simulink model "t_drone"  (R2025b)
settings: Solver=ode23t  StartTime=0.0  StopTime=timespot_spl(end)+2  FixedStep=0.01  MaxStep=1e-2  MinStep=1e-13  RelTol=1e-3  AbsTol=1e-3
InitFcn:
  | model = gcs;
  | 
  | configs = evalin('base', get_param([model '/Configurations'], 'Value'));
  | hold_time = evalin('base', get_param([model '/Hold Time'], 'Value'));
  | transistion_time = evalin('base', get_param([model '/Transistion Time'], 'Value'));
  | 
  | if exist('transforms', 'var') == 1
  |     transforms = transforms;
  | else
  |     transforms = false;
  | end
  | 
  | set_drone_configurations
model workspace (MATLAB code in the model file):
  | load('xy_data_membrane.mat');
undefined symbols (not defined in the file): air_rho, battery, drone_leg, filtD_altitude, filtD_attitude, filtD_motor, filtD_pitch, filtD_position, filtD_roll, filtD_yaw, filtM_altitude, filtM_attitude, filtM_pitch, filtM_position, filtM_roll, filtM_yaw, filtSpd_motor, kd_altitude, kd_attitude, kd_motor, kd_pitch, kd_position, kd_roll, kd_yaw, ki_altitude, ki_attitude, ki_motor, ki_pitch, ki_position, ki_roll, ki_yaw, kp_altitude, kp_attitude, kp_motor, kp_pitch, kp_position, kp_roll, kp_yaw, limit_altitude, limit_attitude, limit_motor, limit_pitch, limit_roll, limit_yaw, mass, pkgDensity, pkgSize, planedepth, pos2attitude, propeller, qc_motor, qd_area, qd_drag, spline_data, spline_yaw, timespot_spl, timespots, waypoints, wind_speed, X ... (+2)
libraries: sm_lib x176, nesl_utility x46, fl_lib x37, slpidlib x9, ee_lib x5, simulink_extras x4, sdl_lib x4, simulink x2, batteryecm_lib x1
(part 1 of 8)
CloseFcn:
  | try,close(h1_quadcopter_package_delivery),end
  | clear h1_quadcopter_package_delivery
  | try,close(h2_quadcopter_package_delivery),end
  | clear h2_quadcopter_package_delivery
  | try,close(h3_quadcopter_package_delivery),end
  | clear h3_quadcopter_package_delivery
  | try,close(h4_quadcopter_package_delivery),end
  | clear h4_quadcopter_package_delivery
Description:
  | Quadcopter Package Delivery
  | Copyright 2021-2025 The MathWorks, Inc.
settings Model: VariantFading=off  Creator=tianwang  LastModifiedBy=Admin
settings SolverCC: AutoScaleAbsTol=off  MaxConsecutiveMinStep=100  AlgebraicLoopSolver=TrustRegion  SolverResetMethod=Robust
settings DataIOCC: MaxDataPoints=10000  ReturnWorkspaceOutputs=off  SignalLoggingName=logsout_quadcopter_package_delivery
settings OptimizationCC: ReuseModelBlockBuffer=off
settings DebuggingCC: ParameterPrecisionLossMsg=none  UnconnectedInputMsg=warning  UnconnectedOutputMsg=warning  UnconnectedLineMsg=warning
settings ModelReferenceCC: EnableRefExpFcnMdlSchedulingChecks=on
settings SFSimCC: CustomCodeUndefinedFunction=UseInterfaceOnly
settings RTWCC: GPUComputeCapability=3.5  DLArmComputeVersion=19.05
settings SimscapeCC: ExplicitSolverDiagnosticOptions=none  SimscapeLogType=all  SimscapeLogSimulationStatistics=on  SimscapeLogToSDI=on  SimscapeLogName=simlog_quadcopter_package_delivery  SimscapeLogLimitData=off  SimscapeLogDataHistory=50000.0
settings DiagnosticsConfigSet: SimMechanicsConflictingReferenceFrames=none  SimMechanicsRigidlyBoundBlock=none
settings ExplorerConfigSet: InternalSimMechanicsExplorerSettings=|
  | <ExplorerConfiguration>
  | 
  |   <canonicalview>default</canonicalview>
  | 
  |   <TilePanel>
  |     <TileInfo>
  |       <Tiles Columns="2" Count="4" Height="692" Rows="2" Width="984">
  |         <Row Weight="0.3531"/>
  |         <Row Weight="0.6469"/>
  |         <Column Weight="0.5664"/>
  |         <Column Weight="0.4336"/>
  |         <Tile Height="1" Width="1" X="0" Y="0"/>
  |         <Tile Height="1" Width="1" X="0" Y="1"/>
  |         <Tile Height="1" Width="1" X="1" Y="0"/>
  |         <Tile Height="1" Width="1" X="1" Y="1"/>
  |       </Tiles>
  |     </TileInfo>
  |     <SceneInfo>
  |       <SceneViewer>
  |         <IsThisViewStd>
  |           <IsStandardView>off</IsStandardView>
  |           <StandardViewName>Front</StandardViewName>
  |         </IsThisViewStd>
  |         <BGColor>
  |           <R>1</R>
  |           <G>1</G>
  |           <B>1</B>
  |           <A>1</A>
  |         </BGColor>
  |         <Camera>
  |           <DoPerspective>on</DoPerspective>
  |           <Position>
  |             <X>3.0099100000000001</X>
  |             <Y>2.9750999999999999</Y>
  |             <Z>0.14957999999999999</Z>
  |           </Position>
  |           <Center>
  |             <X>3.0099100000000001</X>
  |             <Y>3.9750999999999999</Y>
  |             <Z>0.14957999999999999</Z>
  |           </Center>
  |           <Up>
  |             <X>0</X>
  |             <Y>0</Y>
  |             <Z>1</Z>
  |           </Up>
  |           <XLim>0.46630765815499858</XLim>
  |           <YLim>0.46630765815499858</YLim>
  |           <ViewLimDist>0.01</ViewLimDist>
  |         </Camera>
  |       </SceneViewer>
  |       <SceneViewer>
  |         <IsThisViewStd>
  |           <IsStandardView>off</IsStandardView>
  |           <StandardViewName>Front</StandardViewName>
  |         </IsThisViewStd>
  |         <BGColor>
  |           <R>1</R>
  |           <G>1</G>
  |           <B>1</B>
  |           <A>1</A>
  |         </BGColor>
  |         <Camera>
  |           <DoPerspective>on</DoPerspective>
  |           <Position>
  |             <X>3.0099100000000001</X>
  |             <Y>3.9750999999999999</Y>
  |             <Z>1.14958</Z>
  |           </Position>
  |           <Center>
  |             <X>3.0099100000000001</X>
  |             <Y>3.9750999999999999</Y>
  |             <Z>0.14957999999999999</Z>
  |           </Center>
  |           <Up>
  |             <X>0</X>
  |             <Y>1</Y>
  |             <Z>0</Z>
  |           </Up>
  |           <XLim>0.46630765815499869</XLim>
  |           <YLim>0.46630765815499869</YLim>
  |           <ViewLimDist>0.01</ViewLimDist>
  |         </Camera>
  |       </SceneViewer>
  |       <SceneViewer>
  |         <IsThisViewStd>
  |           <IsStandardView>off</IsStandardView>
  |           <StandardViewName>Front</StandardViewName>
  |         </IsThisViewStd>
  |         <BGColor>
  |           <R>1</R>
  |           <G>1</G>
  |           <B>1</B>
  |           <A>1</A>
  |         </BGColor>
  |         <Camera>
  |           <DoPerspective>on</DoPerspective>
  |           <Position>
  |             <X>3.0133399999999999</X>
  |             <Y>4.0542999999999996</Y>
  |             <Z>0.21107000000000001</Z>
  |           </Position>
  |           <Center>
  |             <X>3.04318</X>
  |             <Y>5.0538499999999997</Y>
  |             <Z>0.21099999999999999</Z>
  |           </Center>
  |           <Up>
  |             <X>9.6937670845227242e-06</X>
  |             <Y>6.9742121771481852e-05</Y>
  |             <Z>0.99999999752103363</Z>
  |           </Up>
  |           <XLim>0.46630765815499881</XLim>
  |           <YLim>0.46630765815499881</YLim>
  |           <ViewLimDist>0.01</ViewLimDist>
  |         </Camera>
  |       </SceneViewer>
  |       <SceneViewer>
  |         <IsThisViewStd>
  |           <IsStandardView>off</IsStandardView>
  |           <StandardViewName>Front</StandardViewName>
  |         </IsThisViewStd>
  |         <BGColor>
  |           <R>1</R>
  |           <G>1</G>
  |           <B>1</B>
  |           <A>1</A>
  |         </BGColor>
  |         <Camera>
  |           <DoPerspective>on</DoPerspective>
  |           <Position>
  |             <X>3.5099100000000001</X>
  |             <Y>2.9750999999999999</Y>
  |             <Z>1.14958</Z>
  |           </Position>
  |           <Center>
  |             <X>3.17658</X>
  |             <Y>3.6417600000000001</Y>
  |             <Z>0.48291000000000001</Z>
  |           </Center>
  |           <Up>
  |             <X>-0.29814488151994684</X>
  |             <Y>0.59628976303989367</Y>
  |             <Z>0.74535102342271209</Z>
  |           </Up>
  |           <XLim>0.46630765815499842</XLim>
  |           <YLim>0.46630765815499842</YLim>
  |           <ViewLimDist>0.01</ViewLimDist>
  |         </Camera>
  |       </SceneViewer>
  |     </SceneInfo>
  |   </TilePanel>
  | 
  |   <MechEditorPanel>
  |     <GfxPanelCameraMap>
  |       <MapElement CameraMLId="Camera2" GfxPanelIndex="0"/>
  |       <MapElement CameraMLId="Camera1" GfxPanelIndex="1"/>
  |       <MapElement CameraMLId="Camera6" GfxPanelIndex="2"/>
  |       <MapElement CameraMLId="Camera4" GfxPanelIndex="3"/>
  |     </GfxPanelCameraMap>
  |     <Cameras>
  |       <Camera>
  |         <Id>Camera1</Id>
  |         <Value>
  |           <Name>FixO Top</Name>
  |           <NativeCamera>
  |             <PositionTrackingFeature>Quadcopter.Camera.Cam_FixO_Top.R</PositionTrackingFeature>
  |             <CenterTrackingFeature>Quadcopter.Camera.Cam_FixO_Top.R</CenterTrackingFeature>
  |             <UpVectorTrackingFeature>Quadcopter.Camera.Cam_FixO_Top.R</UpVectorTrackingFeature>
  |             <CenterTrackingOrigin>off</CenterTrackingOrigin>
  |             <CenterTrackingDirection>+X</CenterTrackingDirection>
  |             <UpVectorTrackingDirection>+Y</UpVectorTrackingDirection>
  |           </NativeCamera>
  |         </Value>
  |       </Camera>
  |       <Camera>
  |         <Id>Camera2</Id>
  |         <Value>
  |           <Name>FixO L</Name>
  |           <NativeCamera>
  |             <PositionTrackingFeature>Quadcopter.Camera.Cam_FixO_L.R</PositionTrackingFeature>
  |             <CenterTrackingFeature>Quadcopter.Camera.Cam_FixO_L.R</CenterTrackingFeature>
  |             <UpVectorTrackingFeature>Quadcopter.Camera.Cam_FixO_L.R</UpVectorTrackingFeature>
  |             <CenterTrackingOrigin>off</CenterTrackingOrigin>
  |             <CenterTrackingDirection>+X</CenterTrackingDirection>
  |             <UpVectorTrackingDirection>+Z</UpVectorTrackingDirection>
  |           </NativeCamera>
  |         </Value>
  |       </Camera>
  |       <Camera>
  |         <Id>Camera3</Id>
  |         <Value>
  |           <Name>FixO F</Name>
  |           <NativeCamera>
  |             <PositionTrackingFeature>Quadcopter.Camera.Cam_FixO_F.R</PositionTrackingFeature>
  |             <CenterTrackingFeature>Quadcopter.Camera.Cam_FixO_F.R</CenterTrackingFeature>
  |             <UpVectorTrackingFeature>Quadcopter.Camera.Cam_FixO_F.R</UpVectorTrackingFeature>
  |             <CenterTrackingOrigin>off</CenterTrackingOrigin>
  |             <CenterTrackingDirection>+X</CenterTrackingDirection>
  |             <UpVectorTrackingDirection>+Z</UpVectorTrackingDirection>
  |           </NativeCamera>
  |         </Value>
  |       </Camera>
  |       <Camera>
  |         <Id>Camera4</Id>
  |         <Value>
  |           <Name>FixO UFL</Name>
  |           <NativeCamera>
  |             <PositionTrackingFeature>Quadcopter.Camera.Cam_FixO_UFL.R</PositionTrackingFeature>
  |             <CenterTrackingFeature>Quadcopter.Camera.Cam_FixO_UFL.R</CenterTrackingFeature>
  |             <UpVectorTrackingFeature>Quadcopter.Camera.Cam_FixO_UFL.R</UpVectorTrackingFeature>
  |             <CenterTrackingOrigin>off</CenterTrackingOrigin>
  |             <CenterTrackingDirection>+X</CenterTrackingDirection>
  |             <UpVectorTrackingDirection>+Z</UpVectorTrackingDirection>
  |           </NativeCamera>
  |         </Value>
  |       </Camera>
  |       <Camera>
  |         <Id>Camera5</Id>
  |         <Value>
  |           <Name>Track_Target</Name>
  |           <NativeCamera>
  |             <PositionTrackingFeature>Quadcopter.Camera.Cam_Target.R</PositionTrackingFeature>
  |             <CenterTrackingFeature>Quadcopter.Camera.Transform_Target.F</CenterTrackingFeature>
  |             <UpVectorTrackingFeature>Quadcopter.Camera.Transform_Target.F</UpVectorTrackingFeature>
  |             <CenterTrackingOrigin>on</CenterTrackingOrigin>
  |             <UpVectorTrackingDirection>+Z</UpVectorTrackingDirection>
  |           </NativeCamera>
  |         </Value>
  |       </Camera>
  |       <Camera>
  |         <Id>Camera6</Id>
  |         <Value>
  |           <Name>Track Body Forward</Name>
  |           <NativeCamera>
  |             <PositionTrackingFeature>Quadcopter.Body.Body.Cam_Body_Front.R</PositionTrackingFeature>
  |             <CenterTrackingFeature>Quadcopter.Body.Body.Cam_Body_Front.R</CenterTrackingFeature>
  |             <UpVectorTrackingFeature>Quadcopter.Body.Body.Cam_Body_Front.R</UpVectorTrackingFeature>
  |             <CenterTrackingOrigin>off</CenterTrackingOrigin>
  |             <CenterTrackingDirection>+X</CenterTrackingDirection>
  |             <UpVectorTrackingDirection>+Z</UpVectorTrackingDirection>
  |           </NativeCamera>
  |         </Value>
  |       </Camera>
  |     </Cameras>
  |     <VideoCreator>
  |       <IncludeTiles>All</IncludeTiles>
  |       <IncludeTime>on</IncludeTime>
  |       <IncludeWorldFrame>off</IncludeWorldFrame>
  |       <PlaybackSpeedRatio>1</PlaybackSpeedRatio>
  |       <FrameRate>60</FrameRate>
  |       <FrameSize>[1920, 1080]</FrameSize>
  |       <VideoFormat>UncompressedAVI</VideoFormat>
  |     </VideoCreator>
  |   </MechEditorPanel>
  | 
  |   <PlaybackSettings>
  |     <PlaybackSpeedFactor>2</PlaybackSpeedFactor>
  |   </PlaybackSettings>
  | 
  | </ExplorerConfiguration>

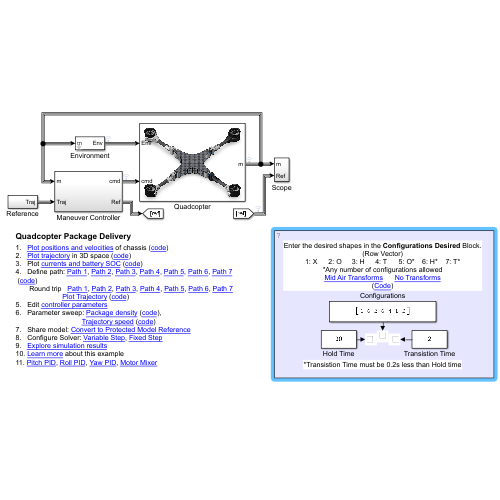
[thumbnail: Simulink's stored preview of the top-level diagram]
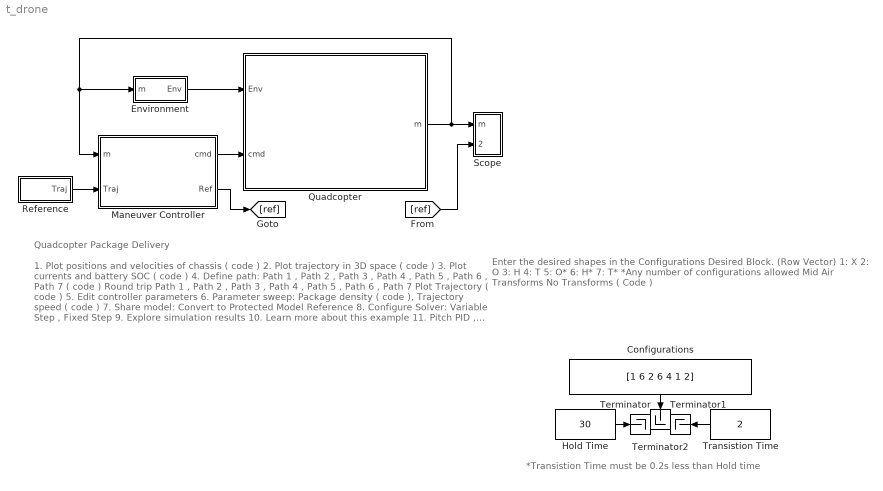
== system t_drone ==
  note: *Transistion Time must be 0.2s less than Hold time
  note: Enter the desired shapes in the Configurations Desired Block.
      | (Row Vector)
      | 1: X 2: O 3: H 4: T 5: O* 6: H* 7: T*
      | *Any number of configurations allowed
      | Mid Air Transforms No Transforms
      | ( Code )
  note: Quadcopter Package Delivery
  note: 1. Plot positions and velocities of chassis ( code )
      | 2. Plot trajectory in 3D space ( code )
      | 3. Plot currents and battery SOC ( code )
      | 4. Define path: Path 1 , Path 2 , Path 3 , Path 4 , Path 5 , Path 6 , Path 7
      | ( code )
      | Round trip Path 1 , Path 2 , Path 3 , Path 4 , Path 5 , Path 6 , Path 7
      | Plot Trajectory ( code )
      | 5. Edit controller parameters
      | 6. Parameter sweep: Package density ( code ),
      | Trajectory speed ( code )
      | 7. Share model: Convert to Protected Model Reference
      | 8. Configure Solver: Variable Step , Fixed Step
      | 9. Explore simulation results
      | 10. Learn more about this example
      | 11. Pitch PID , Roll PID , Yaw PID , Motor Mixer
  Configurations : Constant  Value=[1 6 2 6 4 1 2]
  Environment : Subsystem  mask{wind_speed_mag=wind_speed, height_max_wind=6, height_min_wind=2}
      mask prompts: wind_speed_mag "Wind Speed for Gust (m/s)"; height_max_wind "Lowest Height for Max Wind (m)"; height_min_wind "Maximum Height for Zero Wind (m)"
  Hold Time : Constant  Value=30
  Maneuver Controller : Subsystem
  Quadcopter : Subsystem
      mask Display:
      | %image('quadcopter_body_arms_load.png');
      | image('quadcopter_body_arms_load_basket.png');
  Reference : Subsystem
  Scope : Subsystem
  Terminator : Terminator
  Terminator1 : Terminator
  Terminator2 : Terminator
  Transistion Time : Constant  Value=2
  wires:
  Maneuver Controller/1(cmd) -> Quadcopter/2(cmd)
  Quadcopter/1(m) -> Maneuver Controller/1(m), Environment/1(m), Scope/1(m)
  Reference/1(Traj) -> Maneuver Controller/2(Traj)
  [ref] -> Scope/2(Ref)
  Maneuver Controller/2(Ref) -> [ref]
  Environment/1(Env) -> Quadcopter/1(Env)
  Hold Time/1 -> Terminator/1
  Transistion Time/1 -> Terminator1/1
  Configurations/1 -> Terminator2/1

== system t_drone/Environment ==
  In Bus Element : Inport  PortName=m  Element=Chassis.pz
  Bias Height Min Wind : Bias  Bias=-height_min_wind  SaturateOnIntegerOverflow=off
  Bus Creator2 : BusCreator  Inputs=1
  Constant1 : Constant  Value=0
  Mux1 : Mux  Inputs=3
  Product1 : Product
  Pulse Generator2 : DiscretePulseGenerator  PulseType=Time based  Amplitude=wind_speed_mag  Period=10  PulseWidth=25  PhaseDelay=5
  Pulse Generator3 : DiscretePulseGenerator  PulseType=Time based  Amplitude=wind_speed_mag  Period=10  PulseWidth=25  PhaseDelay=9
  Saturation : Saturate  UpperLimit=height_max_wind-height_min_wind  LowerLimit=0  ZeroCross=off
  "Scale Wind by Height " : Gain  Gain=1/(height_max_wind-height_min_wind)
  Vec to Bus : Subsystem
  Env : Outport
  wires:
  In Bus Element/1 -> Bias Height Min Wind/1
  Bias Height Min Wind/1 -> Saturation/1
  Saturation/1 -> "Scale Wind by Height "/1
  "Scale Wind by Height "/1 -> Product1/1
  Constant1/1 -> Mux1/3  "vz"
  Pulse Generator3/1 -> Mux1/2  "vy"
  Pulse Generator2/1 -> Mux1/1  "vx"
  Mux1/1 -> Product1/2  "wind"
  Product1/1 -> Vec to Bus/1(V)  "wind"
  Vec to Bus/1(B) -> Bus Creator2/1
  Bus Creator2/1 -> Env/1  "Env"

== system t_drone/Maneuver Controller ==
  In Bus Element13 : Inport  PortName=m
  In Bus Element3 : Inport  Port=2  PortName=Traj
  Altitude and YPR Control : Subsystem  mask{attitude_filtM=filtM_attitude, attitude_kp=kp_attitude, attitude_ki=ki_attitude, attitude_kd=kd_attitude, attitude_f=filtD_attitude, attitude_limit=limit_attitude, yaw_filtM=filtM_yaw, yaw_kp=kp_yaw, yaw_ki=ki_yaw, yaw_kd=kd_yaw, yaw_f=filtD_yaw, yaw_limit=limit_yaw, altitude_filtM=filtM_altitude, altitude_kp=kp_altitude, altitude_ki=ki_altitude, altitude_kd=kd_altitude, altitude_f=filtD_altitude, altitude_limit=limit_altitude}
      mask prompts: attitude_filtM "Filter Measurement (s)"; attitude_kp "Kp"; attitude_ki "Ki"; attitude_kd "Kd"; attitude_f "Derivative Filter Coefficient"; attitude_limit "Limit (m/s)"; yaw_filtM "Filter Measurement (s)"; yaw_kp "Kp"; yaw_ki "Ki"; yaw_kd "Kd"; yaw_f "Derivative Filter Coefficient"; yaw_limit "Limit (m/s)"; altitude_filtM "Filter Measurement (s)"; altitude_kp "Kp"; altitude_ki "Ki"; altitude_kd "Kd"; altitude_f "Derivative Filter Coefficient"; altitude_limit "Limit (m/s)"
      mask DialogControl Container3 Prompt: Attitude (Orientation)
      mask DialogControl Container4 Prompt: Yaw
      mask DialogControl Container_alt Prompt: Altitude (Orientation)
  Motor Mixer : Subsystem
  Position Control : Subsystem  mask{filt_pos4attitude=filtM_position, kp_xy2ypr=kp_position, ki_xy2ypr=ki_position, kd_xy2ypr=kd_position, filtD_xy2ypr=filtD_position, err2rp=pos2attitude}
      mask prompts: filt_pos4attitude "Filter Constant (s)"; kp_xy2ypr "Kp"; ki_xy2ypr "Ki"; kd_xy2ypr "Kd"; filtD_xy2ypr "Derivative Filter Coefficient"; err2rp "Position Error to Attitude"
  cmd : Outport
  Ref : Outport  Port=2
  wires:
  Motor Mixer/1(Cmd) -> cmd/1
  Altitude and YPR Control/2(Motor Roll) -> Motor Mixer/2(Roll Cmd)
  Altitude and YPR Control/1(Motor Pitch) -> Motor Mixer/1(Pitch Cmd)
  Altitude and YPR Control/3(Motor Yaw) -> Motor Mixer/3(Yaw Cmd)
  Altitude and YPR Control/4(Motor Thrust) -> Motor Mixer/4(Thrust Cmd)
  Position Control/2(Roll Cmd) -> Altitude and YPR Control/4(Roll Cmd)
  Position Control/1(Pitch Cmd) -> Altitude and YPR Control/3(Pitch Cmd)
  In Bus Element13/1 -> Position Control/1(m), Altitude and YPR Control/1(m)
  In Bus Element3/1 -> Position Control/2(Traj), Altitude and YPR Control/2(Ref)
  Position Control/3(Yaw Cmd) -> Altitude and YPR Control/5(Yaw Cmd)
  Position Control/4(Ref) -> Ref/1

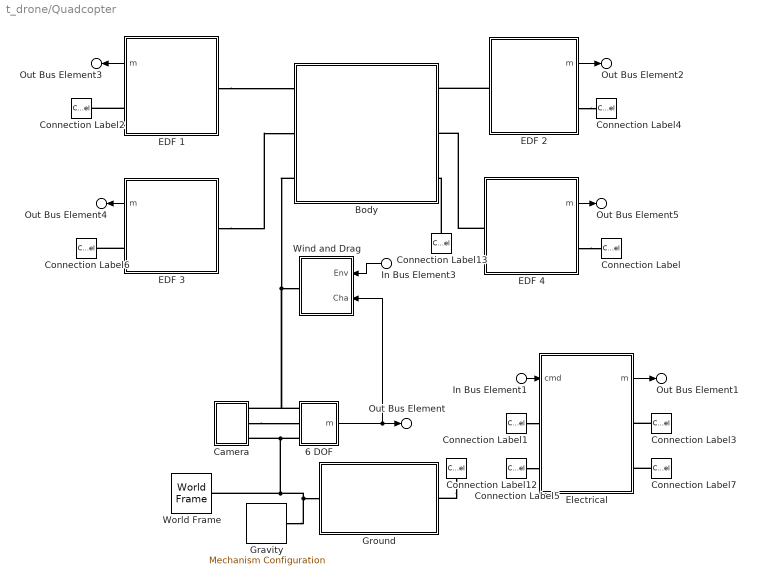
== system t_drone/Quadcopter ==
  In Bus Element3 : Inport  PortName=Env  Element=wind
  In Bus Element1 : Inport  Port=2  PortName=cmd
  6 DOF : Subsystem
  Body : Subsystem
      mask Display: image('quadcopter_body_arms.png');
  Camera : Subsystem
  Connection Label : ConnectionLabel  Label=P4
  Connection Label1 : ConnectionLabel  Label=P4
  Connection Label12 : ConnectionLabel  Label=G
  Connection Label13 : ConnectionLabel  Label=G
  Connection Label2 : ConnectionLabel  Label=P1
  Connection Label3 : ConnectionLabel  Label=P1
  Connection Label4 : ConnectionLabel  Label=P2
  Connection Label5 : ConnectionLabel  Label=P2
  Connection Label6 : ConnectionLabel  Label=P3
  Connection Label7 : ConnectionLabel  Label=P3
  EDF 1 : Subsystem  mask{popup_prop_pos=1 or 4}
      mask prompts: popup_prop_pos "Propeller Position"
      mask init:
      | if(strcmp(get_param(gcb,'popup_prop_pos'),'1 or 4'))
      |     set_param([gcb '/Propeller'],'ExtGeomFileName','quadcopter_drone_12_blade_fans.stp');
      |     set_param([gcb '/Thrust Direction'],'Gain','1');
      | else
      |     set_param([gcb '/Propeller'],'ExtGeomFileName','quadcopter_drone_12_blade_fans.stp');
      |     set_param([gcb '/Thrust Direction'],'Gain','-1');
      | end
      mask TypeOptions popup_prop_pos: 1 or 4 | 2 or 3
      mask Display:
      | if(strcmp(get_param(gcb,'popup_prop_pos'),'1 or 4'))
      |     image('quadcopter_motor_prop_1_4.png');
      | else
      |     image('quadcopter_motor_prop_2_3.png');
      | end
  EDF 2 : Subsystem  mask{popup_prop_pos=2 or 3}
      mask prompts: popup_prop_pos "Propeller Position"
      mask init: same as t_drone/Quadcopter/EDF 1
      mask TypeOptions popup_prop_pos: 1 or 4 | 2 or 3
      mask Display:
      | if(strcmp(get_param(gcb,'popup_prop_pos'),'1 or 4'))
      |     image('quadcopter_motor_prop_1_4.png');
      | else
      |     image('quadcopter_motor_prop_2_3.png');
      | end
  EDF 3 : Subsystem  mask{popup_prop_pos=2 or 3}
      mask prompts: popup_prop_pos "Propeller Position"
      mask init: same as t_drone/Quadcopter/EDF 1
      mask TypeOptions popup_prop_pos: 1 or 4 | 2 or 3
      mask Display:
      | if(strcmp(get_param(gcb,'popup_prop_pos'),'1 or 4'))
      |     image('quadcopter_motor_prop_1_4.png');
      | else
      |     image('quadcopter_motor_prop_2_3.png');
      | end
  EDF 4 : Subsystem  mask{popup_prop_pos=1 or 4}
      mask prompts: popup_prop_pos "Propeller Position"
      mask init: same as t_drone/Quadcopter/EDF 1
      mask TypeOptions popup_prop_pos: 1 or 4 | 2 or 3
      mask Display:
      | if(strcmp(get_param(gcb,'popup_prop_pos'),'1 or 4'))
      |     image('quadcopter_motor_prop_1_4.png');
      | else
      |     image('quadcopter_motor_prop_2_3.png');
      | end
  Electrical : Subsystem  mask{trq_max=qc_motor.max_torque, power_max=qc_motor.max_power, trq_tc=qc_motor.time_const, eff_overall=qc_motor.efficiency, eff_spd=qc_motor.efficiency_spd, eff_trq=qc_motor.efficiency_trq, rotor_d=qc_motor.rotor_damping, kp=kp_motor, ki=ki_motor, kd=kd_motor, f_deriv=filtD_motor, f_spd=filtSpd_motor, max_trq_cmd=limit_motor}
      mask prompts: trq_max "Max Torque (N*m)"; power_max "Max Power (W)"; trq_tc "Time Constant, Torque (s)"; eff_overall "Efficiency (%)"; eff_spd "Speed for Efficiency (rpm)"; eff_trq "Torque for Efficiency (N*m)"; rotor_d "Rotor Damping (N*m/(rad/s))"; kp "Proportional"; ki "Integral"; kd "Derivative"; f_deriv "Filter on Error Derivative (N)"; f_spd "Filter on Speed Measurement (sec)"; max_trq_cmd "Saturation (N*m)"
      mask DialogControl Container4 Prompt: Motor
      mask DialogControl Container9 Prompt: Control
      mask Display: image('quadcopter_electric.png');
  Gravity : sm_lib/Utilities/Mechanism Configuration  UniformGravity=Constant  GravityVector=[0 0 -9.80665]  GravityVectorUnits=m/s^2  LinearizationDelta=0.001  JointModeTransitionNonlinearIterations=2
  Ground : Subsystem
      mask Display: image('ground_launch_target.PNG');
  Wind and Drag : Subsystem
  World Frame : sm_lib/Frames and Transforms/World Frame
  Out Bus Element : Outport  PortName=m  Element=Chassis
  Out Bus Element1 : Outport  PortName=m  Element=Motor
  Out Bus Element2 : Outport  PortName=m  Element=Prop2
  Out Bus Element3 : Outport  PortName=m  Element=Prop1
  Out Bus Element4 : Outport  PortName=m  Element=Prop3
  Out Bus Element5 : Outport  PortName=m  Element=Prop4
  wires:
  EDF 4/1(m) -> Out Bus Element5/1
  EDF 1/1(m) -> Out Bus Element3/1
  EDF 3/1(m) -> Out Bus Element4/1
  Electrical/1(m) -> Out Bus Element1/1
  EDF 2/1(m) -> Out Bus Element2/1
  In Bus Element1/1 -> Electrical/1(cmd)
  6 DOF/1(m) -> Out Bus Element/1, Wind and Drag/2(Cha)
  In Bus Element3/1 -> Wind and Drag/1(Env)
  connections:
  Body/LConn3 -- 6 DOF/LConn1 -- Camera/RConn1 -- Wind and Drag/RConn1
  EDF 2/LConn1 -- Body/RConn1
  EDF 1/LConn1 -- Body/LConn1
  EDF 4/LConn1 -- Body/RConn2
  EDF 3/LConn1 -- Body/LConn2
  Connection Label13/LConn1 -- Body/RConn3
  EDF 4/RConn1 -- Connection Label/LConn1
  Connection Label1/LConn1 -- Electrical/LConn1
  EDF 1/RConn1 -- Connection Label2/LConn1
  Connection Label3/LConn1 -- Electrical/RConn1
  EDF 2/RConn1 -- Connection Label4/LConn1
  Connection Label5/LConn1 -- Electrical/LConn2
  EDF 3/RConn1 -- Connection Label6/LConn1
  Connection Label7/LConn1 -- Electrical/RConn2
  Gravity/RConn1 -- 6 DOF/LConn3 -- Camera/RConn3 -- World Frame/RConn1 -- Ground/RConn1
  Connection Label12/LConn1 -- Ground/LConn1
  Camera/RConn2 -- 6 DOF/LConn2

== system t_drone/Reference ==
  Clock1 : Clock
  Derivative : Subsystem
  Interpolate Spline Points : Subsystem
  Out Bus Element : Outport  PortName=Traj  Element=pos
  Out Bus Element1 : Outport  PortName=Traj  Element=vel
  Out Bus Element2 : Outport  PortName=Traj  Element=yaw
  wires:
  Clock1/1 -> Interpolate Spline Points/1(In1)
  Interpolate Spline Points/2(des_pos) -> Out Bus Element/1, Derivative/1(des xyz)
  Interpolate Spline Points/1(Yaw) -> Out Bus Element2/1
  Derivative/1(des_vel) -> Out Bus Element1/1

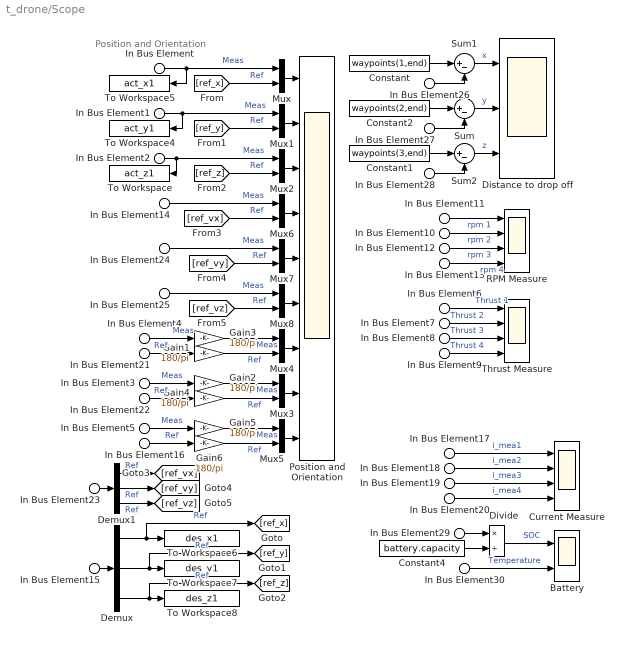
== system t_drone/Scope ==
  note: Position and Orientation
  In Bus Element : Inport  PortName=m  Element=Chassis.px
  In Bus Element26 : Inport  PortName=m  Element=Chassis.px
  In Bus Element1 : Inport  PortName=m  Element=Chassis.py
  In Bus Element27 : Inport  PortName=m  Element=Chassis.py
  In Bus Element2 : Inport  PortName=m  Element=Chassis.pz
  In Bus Element28 : Inport  PortName=m  Element=Chassis.pz
  In Bus Element3 : Inport  PortName=m  Element=Chassis.pitch
  In Bus Element4 : Inport  PortName=m  Element=Chassis.roll
  In Bus Element5 : Inport  PortName=m  Element=Chassis.yaw
  In Bus Element14 : Inport  PortName=m  Element=Chassis.vx
  In Bus Element24 : Inport  PortName=m  Element=Chassis.vy
  In Bus Element25 : Inport  PortName=m  Element=Chassis.vz
  In Bus Element7 : Inport  PortName=m  Element=Prop2.thrust
  In Bus Element10 : Inport  PortName=m  Element=Prop2.w
  In Bus Element6 : Inport  PortName=m  Element=Prop1.thrust
  In Bus Element11 : Inport  PortName=m  Element=Prop1.w
  In Bus Element8 : Inport  PortName=m  Element=Prop3.thrust
  In Bus Element12 : Inport  PortName=m  Element=Prop3.w
  In Bus Element9 : Inport  PortName=m  Element=Prop4.thrust
  In Bus Element13 : Inport  PortName=m  Element=Prop4.w
  In Bus Element17 : Inport  PortName=m  Element=Motor.Mot1.i
  In Bus Element18 : Inport  PortName=m  Element=Motor.Mot2.i
  In Bus Element19 : Inport  PortName=m  Element=Motor.Mot3.i
  In Bus Element20 : Inport  PortName=m  Element=Motor.Mot4.i
  In Bus Element29 : Inport  PortName=m  Element=Motor.Battery.SOC
  In Bus Element30 : Inport  PortName=m  Element=Motor.Battery.degC
  In Bus Element15 : Inport  Port=2  PortName=Ref  Element=pos
  In Bus Element16 : Inport  Port=2  PortName=Ref  Element=yaw
  In Bus Element21 : Inport  Port=2  PortName=Ref  Element=roll
  In Bus Element22 : Inport  Port=2  PortName=Ref  Element=pitch
  In Bus Element23 : Inport  Port=2  PortName=Ref  Element=vel
  Battery : Scope  NumInputPorts=2
      settings: ActiveDisplayYMinimum=0.99219  ActiveDisplayYMaximum=1.00087
  Constant : Constant  Value=waypoints(1,end)
  Constant1 : Constant  Value=waypoints(3,end)
  Constant2 : Constant  Value=waypoints(2,end)
  Constant4 : Constant  Value=battery.capacity
  Current Measure : Scope  NumInputPorts=4
      settings: ActiveDisplayYMinimum=-5.48055  ActiveDisplayYMaximum=19.1285  DataLoggingVariableName=ScopeData2
  Demux : Demux  Outputs=3
  Demux1 : Demux  Outputs=3
  Distance to drop off : Scope  NumInputPorts=3
      settings: ActiveDisplayYMinimum=-0.83846  ActiveDisplayYMaximum=0.45879
  Divide : Product  Inputs=*/
  Gain{1..6} (6 alike) : Gain  Gain=180/pi
  Mux{,1..8} (9 alike) : Mux  Inputs=2
  Position and Orientation : Scope  NumInputPorts=9
      settings: Title=px  ActiveDisplayYMinimum=-2.95256  ActiveDisplayYMaximum=5.99591  DataLoggingVariableName=ScopeData2
  RPM Measure : Scope  NumInputPorts=4
      settings: ActiveDisplayYMinimum=-7347.52347  ActiveDisplayYMaximum=7432.06356  DataLoggingVariableName=ScopeData2
  Sum : Sum  Inputs=|+-
  Sum1 : Sum  Inputs=|+-
  Sum2 : Sum  Inputs=|+-
  Thrust Measure : Scope  NumInputPorts=4
      settings: ActiveDisplayYMinimum=-0.67587  ActiveDisplayYMaximum=6.05582
  To Workspace : ToWorkspace  VariableName=act_z1  SampleTime=-1
  To Workspace4 : ToWorkspace  VariableName=act_y1  SampleTime=-1
  To Workspace5 : ToWorkspace  VariableName=act_x1  SampleTime=-1
  To Workspace6 : ToWorkspace  VariableName=des_x1  SampleTime=-1
  To Workspace7 : ToWorkspace  VariableName=des_y1  SampleTime=-1
  To Workspace8 : ToWorkspace  VariableName=des_z1  SampleTime=-1
  wires:
  In Bus Element7/1 -> Thrust Measure/2  "Thrust 2"
  In Bus Element9/1 -> Thrust Measure/4  "Thrust 4"
  In Bus Element8/1 -> Thrust Measure/3  "Thrust 3"
  In Bus Element6/1 -> Thrust Measure/1  "Thrust 1"
  In Bus Element11/1 -> RPM Measure/1  "rpm 1"
  In Bus Element10/1 -> RPM Measure/2  "rpm 2"
  In Bus Element12/1 -> RPM Measure/3  "rpm 3"
  In Bus Element13/1 -> RPM Measure/4  "rpm 4"
  Demux/3 -> [ref_z], To Workspace8/1  "Ref"
  In Bus Element2/1 -> Mux2/1, To Workspace/1  "Meas"
  In Bus Element17/1 -> Current Measure/1  "i_mea1"
  In Bus Element18/1 -> Current Measure/2  "i_mea2"
  In Bus Element19/1 -> Current Measure/3  "i_mea3"
  In Bus Element20/1 -> Current Measure/4  "i_mea4"
  Gain2/1 -> Mux3/1  "Meas"
  Gain3/1 -> Mux4/1  "Meas"
  Gain5/1 -> Mux5/1  "Meas"
  Demux/2 -> [ref_y], To Workspace7/1  "Ref"
  In Bus Element1/1 -> Mux1/1, To Workspace4/1  "Meas"
  Demux/1 -> To Workspace6/1, [ref_x]  "Ref"
  In Bus Element/1 -> Mux/1, To Workspace5/1  "Meas"
  In Bus Element28/1 -> Sum2/2
  Constant1/1 -> Sum2/1
  Constant2/1 -> Sum/1
  In Bus Element27/1 -> Sum/2
  Constant/1 -> Sum1/1
  In Bus Element26/1 -> Sum1/2
  Sum/1 -> Distance to drop off/2  "y"
  Sum1/1 -> Distance to drop off/1  "x"
  Sum2/1 -> Distance to drop off/3  "z"
  Mux/1 -> Position and Orientation/1
  Mux1/1 -> Position and Orientation/2
  Mux2/1 -> Position and Orientation/3
  Mux3/1 -> Position and Orientation/8
  Mux4/1 -> Position and Orientation/7
  Mux5/1 -> Position and Orientation/9
  In Bus Element15/1 -> Demux/1
  [ref_x] -> Mux/2  "Ref"
  [ref_y] -> Mux1/2  "Ref"
  [ref_z] -> Mux2/2  "Ref"
  In Bus Element23/1 -> Demux1/1
  Demux1/1 -> [ref_vx]  "Ref"
  Demux1/2 -> [ref_vy]  "Ref"
  Demux1/3 -> [ref_vz]  "Ref"
  Mux8/1 -> Position and Orientation/6
  Mux7/1 -> Position and Orientation/5
  Mux6/1 -> Position and Orientation/4
  [ref_vx] -> Mux6/2  "Ref"
  [ref_vy] -> Mux7/2  "Ref"
  [ref_vz] -> Mux8/2  "Ref"
  In Bus Element14/1 -> Mux6/1  "Meas"
  In Bus Element24/1 -> Mux7/1  "Meas"
  In Bus Element25/1 -> Mux8/1  "Meas"
  In Bus Element21/1 -> Gain1/1  "Ref"
  In Bus Element22/1 -> Gain4/1  "Ref"
  In Bus Element16/1 -> Gain6/1  "Ref"
  In Bus Element4/1 -> Gain3/1  "Meas"
  Gain1/1 -> Mux4/2  "Ref"
  In Bus Element3/1 -> Gain2/1  "Meas"
  Gain4/1 -> Mux3/2  "Ref"
  In Bus Element5/1 -> Gain5/1  "Meas"
  Gain6/1 -> Mux5/2  "Ref"
  In Bus Element29/1 -> Divide/1
  Constant4/1 -> Divide/2
  Divide/1 -> Battery/1  "SOC"
  In Bus Element30/1 -> Battery/2  "Temperature"

== system t_drone/Environment/Vec to Bus ==
  V : Inport
  Bus Creator : BusCreator  Inputs=3
  Demux : Demux  Outputs=3
  B : Outport
  wires:
  Demux/3 -> Bus Creator/3  "vz"
  V/1 -> Demux/1
  Demux/1 -> Bus Creator/1  "vx"
  Demux/2 -> Bus Creator/2  "vy"
  Bus Creator/1 -> B/1  "wind"

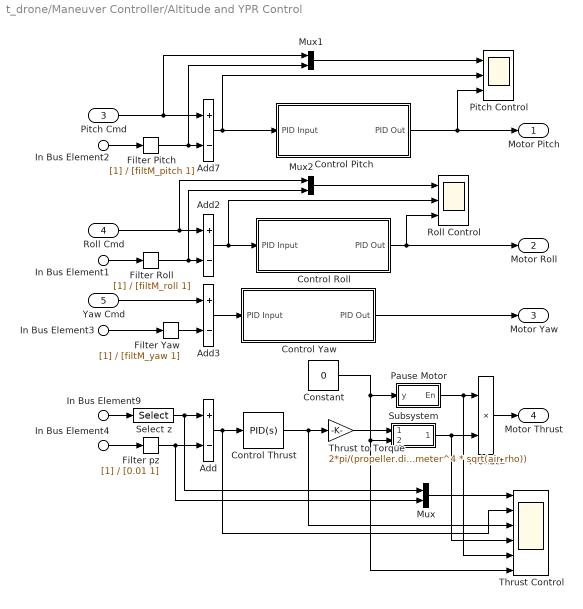
== system t_drone/Maneuver Controller/Altitude and YPR Control ==
  In Bus Element1 : Inport  PortName=m  Element=Chassis.roll
  In Bus Element2 : Inport  PortName=m  Element=Chassis.pitch
  In Bus Element3 : Inport  PortName=m  Element=Chassis.yaw
  In Bus Element4 : Inport  PortName=m  Element=Chassis.pz
  In Bus Element9 : Inport  Port=2  PortName=Ref  Element=pos
  Pitch Cmd : Inport  Port=3
  Roll Cmd : Inport  Port=4
  Yaw Cmd : Inport  Port=5
  Add{,2..3,7} (4 alike) : Sum  Inputs=+-
  Constant : Constant  Value=0
  Control Pitch : Subsystem  mask{ts_p=kp_pitch, ts_i=ki_pitch, ts_d=kd_pitch, ts_f=filtD_pitch, ts_l=limit_pitch, time_spots=timespots}
      mask prompts: ts_p "Proportional"; ts_i "Integral"; ts_d "Derivative"; ts_f "Filter Coefficient"; ts_l "Limit"; time_spots "Time Intervals"
  Control Roll : Subsystem  mask{ts_p=kp_roll, ts_i=ki_roll, ts_d=kd_roll, ts_f=filtD_roll, ts_l=limit_roll, time_spots=timespots}
      mask prompts: ts_p "Proportional"; ts_i "Integral"; ts_d "Derivative"; ts_f "Filter Coefficient"; ts_l "Limit"; time_spots "Time Intervals"
  Control Thrust : slpidlib/PID Controller  Controller=PID  Form=Parallel  TimeDomain=Continuous-time  UseExternalTs=off  SampleTime=-1  IntegratorMethod=Forward Euler  FilterMethod=Forward Euler  ControllerParametersSource=internal  P=altitude_kp  I=altitude_ki  UseKiTs=off  D=altitude_kd  UseExternalDerivativeSource=off  N=altitude_f  UseFilter=on  TunerSelectOption=Transfer Function Based (PID Tuner App)  ZeroCross=off  InitialConditionSource=internal  InitialConditionForIntegrator=0  InitialConditionForFilter=0  DifferentiatorICPrevScaledInput=0  ExternalReset=none  TrackingMode=off  Kt=1  LimitOutput=on  SatLimitsSource=internal  UpperSaturationLimit=altitude_limit  LowerSaturationLimit=-altitude_limit  LinearizeAsGain=on  AntiWindupMode=none  Kb=1  LimitIntegrator=off  UpperIntegratorSaturationLimit=inf  LowerIntegratorSaturationLimit=-inf  POutMin=[]  POutMax=[]  IOutMin=[]  IOutMax=[]  DOutMin=[]  DOutMax=[]  NOutMin=[]  NOutMax=[]  SumOutMin=[]  SumOutMax=[]  SaturationOutMin=[]  SaturationOutMax=[]  PParamMin=[]  PParamMax=[]  IParamMin=[]  IParamMax=[]  DParamMin=[]  DParamMax=[]  NParamMin=[]  NParamMax=[]  KbParamMin=[]  KbParamMax=[]  KtParamMin=[]  KtParamMax=[]  KbOutMin=[]  KbOutMax=[]  KtOutMin=[]  KtOutMax=[]  IntegratorOutMin=[]  IntegratorOutMax=[]  FilterOutMin=[]  FilterOutMax=[]  SumI1OutMin=[]  SumI1OutMax=[]  SumI2OutMin=[]  SumI2OutMax=[]  SumI3OutMin=[]  SumI3OutMax=[]  SumI4OutMin=[]  SumI4OutMax=[]  SumDOutMin=[]  SumDOutMax=[]  DifferentiatorOutMin=[]  DifferentiatorOutMax=[]  FilterDiffOutCoefMin=[]  FilterDiffOutCoefMax=[]  ReciprocalOutMin=[]  ReciprocalOutMax=[]  SumDenOutMin=[]  SumDenOutMax=[]  SumNumOutMin=[]  SumNumOutMax=[]  DivideOutMin=[]  DivideOutMax=[]  UdiffTsProdOutMin=[]  UdiffTsProdOutMax=[]  NTsProdOutMin=[]  NTsProdOutMax=[]  UintegralTsProdOutMin=[]  UintegralTsProdOutMax=[]  UngainTsProdOutMin=[]  UngainTsProdOutMax=[]  ClampingZeroOutDataTypeStr=Inherit: Inherit via back propagation  ClampingZeroOutMin=[]  ClampingZeroOutMax=[]  FilterDenConstantOutDataTypeStr=Inherit: Inherit via back propagation  FilterDenConstantOutMin=[]  FilterDenConstantOutMax=[]  PCopyOutDataTypeStr=Inherit: Inherit via back propagation  PCopyOutMin=[]  PCopyOutMax=[]  NCopyOutDataTypeStr=Inherit: Inherit via back propagation  NCopyOutMin=[]  NCopyOutMax=[]  IntegratorContinuousStateAttributes=''  IntegratorStateMustResolveToSignalObject=off  IntegratorRTWStateStorageClass=Auto  FilterContinuousStateAttributes=''  FilterStateMustResolveToSignalObject=off  FilterRTWStateStorageClass=Auto  ParallelPVariant=InternalParameters  IdealPVariant=Disabled  IVariant=InternalParameters  DVariant=InternalParameters  IntegratorVariant=Continuous  SatVariant=Enabled  AWVariant=Passthrough  PCopyVariant=Disabled  TRVariant=Disabled  FdbkBlocksVariant=Forward  IdealPFdbkVariant=Disabled  SatFdbkVariant=Disabled  DerivativeFilterVariant=ContFilter  NVariant=InternalParameters  NCopyVariant=Disabled  FilterICVariant=InternalICsFilter  IntegratorICVariant=InternalICs  ExternalResetVariant=Disabled  TRSumVariant=Passthrough  SumFdbkVariant=Disabled  SumVariant=Sum_PID  TsampFilterVariant=InternalTs  TsampNgainVariant=Passthrough  TsampIntegralVariant=Disabled_SignalSpec  ExternalSaturationOutDataTypeStr=Inherit: Same as second input  DerivativeSourceVariant=ErrorSignal  PreIntVariant=InternalPreInt
  Control Yaw : Subsystem  mask{ts_p=kp_yaw, ts_i=ki_yaw, ts_d=kd_yaw, ts_f=filtD_yaw, ts_l=limit_yaw, time_spots=timespots}
      mask prompts: ts_p "Proportional"; ts_i "Integral"; ts_d "Derivative"; ts_f "Filter Coefficient"; ts_l "Limit"; time_spots "Time Intervals"
  Filter Pitch : TransferFcn  Denominator=[filtM_pitch 1]
  Filter Roll : TransferFcn  Denominator=[filtM_roll 1]
  Filter Yaw : TransferFcn  Denominator=[filtM_yaw 1]
  Filter pz : TransferFcn  Denominator=[0.01 1]
  Mux : Mux  Inputs=2
  Mux1 : Mux  Inputs=2
  Mux2 : Mux  Inputs=2
  Pause Motor : Subsystem  mask{ts_pulse=0.5, dur_pulse=2}
      mask prompts: ts_pulse "Pulse resolution (sec)"; dur_pulse "Pulse duration (sec)"
  Pitch Control : Scope  NumInputPorts=3
      settings: ActiveDisplayYMinimum=-0.80585  ActiveDisplayYMaximum=0.83815
  Product : Product
  Roll Control : Scope  NumInputPorts=3
      settings: ActiveDisplayYMinimum=-0.80585  ActiveDisplayYMaximum=0.83815
  Select z : Selector  InputPortWidth=3  IndexOptions=Index vector (dialog)  Indices=[3]  OutputSizes=1
  Subsystem : Subsystem
  Thrust Control : Scope  NumInputPorts=6
      settings: ActiveDisplayYMinimum=-0.7525151669788791  ActiveDisplayYMaximum=6.772636502809914  DataLoggingVariableName=ScopeData2
  Thrust to Torque : Gain  Gain=2*pi/(propeller.diameter^4 * sqrt(air_rho))
  Motor Pitch : Outport
  Motor Roll : Outport  Port=2
  Motor Yaw : Outport  Port=3
  Motor Thrust : Outport  Port=4
  wires:
  Pitch Cmd/1 -> Mux1/1, Add7/1
  In Bus Element3/1 -> Filter Yaw/1
  Add7/1 -> Control Pitch/1(PID Input), Pitch Control/2
  Yaw Cmd/1 -> Add3/1
  In Bus Element2/1 -> Filter Pitch/1
  Select z/1 -> Mux/1, Add/1
  In Bus Element1/1 -> Filter Roll/1
  Add3/1 -> Control Yaw/1(PID Input)
  In Bus Element9/1 -> Select z/1
  Add/1 -> Control Thrust/1, Thrust Control/2
  Control Thrust/1 -> Thrust Control/3, Thrust to Torque/1
  Mux/1 -> Thrust Control/1
  Mux1/1 -> Pitch Control/1
  In Bus Element4/1 -> Filter pz/1
  Filter Pitch/1 -> Mux1/2, Add7/2
  Filter Yaw/1 -> Add3/2
  Filter pz/1 -> Mux/2, Add/2
  Product/1 -> Motor Thrust/1
  Pause Motor/1(En) -> Thrust Control/5, Product/1
  Constant/1 -> Pause Motor/1(y), Thrust Control/6, Subsystem/2(load)
  Subsystem/1(Out1) -> Product/2, Thrust Control/4
  Thrust to Torque/1 -> Subsystem/1(cmd)
  Filter Roll/1 -> Mux2/2, Add2/2
  Mux2/1 -> Roll Control/1
  Add2/1 -> Control Roll/1(PID Input), Roll Control/2
  Roll Cmd/1 -> Add2/1, Mux2/1
  Control Pitch/1(PID Out) -> Pitch Control/3, Motor Pitch/1
  Control Roll/1(PID Out) -> Motor Roll/1, Roll Control/3
  Control Yaw/1(PID Out) -> Motor Yaw/1

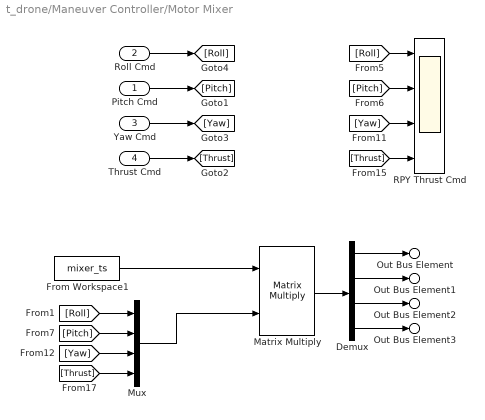
== system t_drone/Maneuver Controller/Motor Mixer ==
  Pitch Cmd : Inport
  Roll Cmd : Inport  Port=2
  Yaw Cmd : Inport  Port=3
  Thrust Cmd : Inport  Port=4
  Demux : Demux
  From Workspace1 : FromWorkspace  VariableName=mixer_ts  OutputAfterFinalValue=Holding final value
  Matrix Multiply : Product  Multiplication=Matrix(*)
  Mux : Mux
  RPY Thrust Cmd : Scope  NumInputPorts=4
      settings: ActiveDisplayYMinimum=4417.97471  ActiveDisplayYMaximum=5987.32527
  Out Bus Element : Outport  PortName=Cmd  Element=w1
  Out Bus Element1 : Outport  PortName=Cmd  Element=w2
  Out Bus Element2 : Outport  PortName=Cmd  Element=w3
  Out Bus Element3 : Outport  PortName=Cmd  Element=w4
  wires:
  Roll Cmd/1 -> [Roll]
  Pitch Cmd/1 -> [Pitch]
  Yaw Cmd/1 -> [Yaw]
  Thrust Cmd/1 -> [Thrust]
  [Roll] -> Mux/1
  [Roll] -> RPY Thrust Cmd/1
  [Pitch] -> RPY Thrust Cmd/2
  [Pitch] -> Mux/2
  [Yaw] -> RPY Thrust Cmd/3
  [Yaw] -> Mux/3
  [Thrust] -> RPY Thrust Cmd/4
  [Thrust] -> Mux/4
  Matrix Multiply/1 -> Demux/1
  Demux/1 -> Out Bus Element/1
  From Workspace1/1 -> Matrix Multiply/1
  Mux/1 -> Matrix Multiply/2
  Demux/2 -> Out Bus Element1/1
  Demux/3 -> Out Bus Element2/1
  Demux/4 -> Out Bus Element3/1

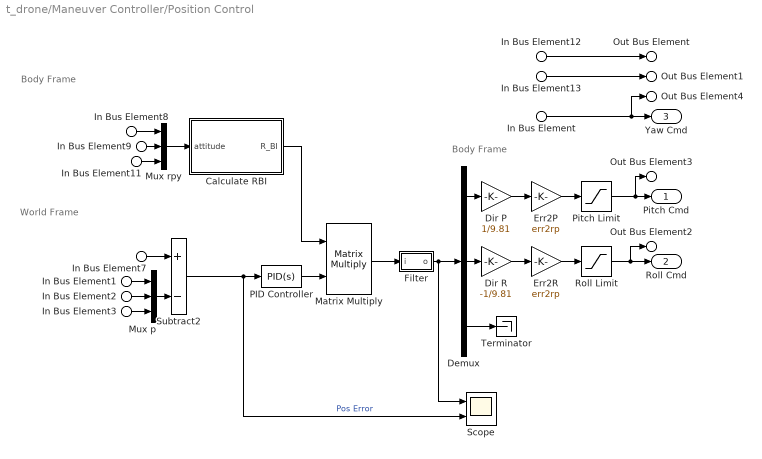
== system t_drone/Maneuver Controller/Position Control ==
  note: Body Frame
  note: World Frame
  note: Body Frame
  In Bus Element1 : Inport  PortName=m  Element=Chassis.px
  In Bus Element2 : Inport  PortName=m  Element=Chassis.py
  In Bus Element3 : Inport  PortName=m  Element=Chassis.pz
  In Bus Element8 : Inport  PortName=m  Element=Chassis.roll
  In Bus Element9 : Inport  PortName=m  Element=Chassis.pitch
  In Bus Element11 : Inport  PortName=m  Element=Chassis.yaw
  In Bus Element7 : Inport  Port=2  PortName=Traj  Element=pos
  In Bus Element12 : Inport  Port=2  PortName=Traj  Element=pos
  In Bus Element13 : Inport  Port=2  PortName=Traj  Element=vel
  In Bus Element : Inport  Port=2  PortName=Traj  Element=yaw
  Calculate RBI : MATLAB Function  TreatAsAtomicUnit=on
  Demux : Demux  Outputs=3
  Dir P : Gain  Gain=1/9.81
  Dir R : Gain  Gain=-1/9.81
  Err2P : Gain  Gain=err2rp
  Err2R : Gain  Gain=err2rp
  Filter : Subsystem  mask{filt_const=filt_pos4attitude}
      mask prompts: filt_const "Filter Constant"
  Matrix Multiply : Product  Multiplication=Matrix(*)
  Mux p : Mux  Inputs=3
  Mux rpy : Mux  Inputs=3
  PID Controller : slpidlib/PID Controller  Controller=PID  Form=Parallel  TimeDomain=Continuous-time  UseExternalTs=off  SampleTime=-1  IntegratorMethod=Forward Euler  FilterMethod=Forward Euler  ControllerParametersSource=internal  P=kp_xy2ypr  I=ki_xy2ypr  UseKiTs=off  D=kd_xy2ypr  UseExternalDerivativeSource=off  N=filtD_xy2ypr  UseFilter=on  TunerSelectOption=Transfer Function Based (PID Tuner App)  InitialConditionSource=internal  InitialConditionForIntegrator=0  InitialConditionForFilter=0  DifferentiatorICPrevScaledInput=0  ExternalReset=none  TrackingMode=off  Kt=1  LimitOutput=off  SatLimitsSource=internal  UpperSaturationLimit=inf  LowerSaturationLimit=-inf  LinearizeAsGain=on  AntiWindupMode=none  Kb=1  LimitIntegrator=off  UpperIntegratorSaturationLimit=inf  LowerIntegratorSaturationLimit=-inf  POutMin=[]  POutMax=[]  IOutMin=[]  IOutMax=[]  DOutMin=[]  DOutMax=[]  NOutMin=[]  NOutMax=[]  SumOutMin=[]  SumOutMax=[]  SaturationOutMin=[]  SaturationOutMax=[]  PParamMin=[]  PParamMax=[]  IParamMin=[]  IParamMax=[]  DParamMin=[]  DParamMax=[]  NParamMin=[]  NParamMax=[]  KbParamMin=[]  KbParamMax=[]  KtParamMin=[]  KtParamMax=[]  KbOutMin=[]  KbOutMax=[]  KtOutMin=[]  KtOutMax=[]  IntegratorOutMin=[]  IntegratorOutMax=[]  FilterOutMin=[]  FilterOutMax=[]  SumI1OutMin=[]  SumI1OutMax=[]  SumI2OutMin=[]  SumI2OutMax=[]  SumI3OutMin=[]  SumI3OutMax=[]  SumI4OutMin=[]  SumI4OutMax=[]  SumDOutMin=[]  SumDOutMax=[]  DifferentiatorOutMin=[]  DifferentiatorOutMax=[]  FilterDiffOutCoefMin=[]  FilterDiffOutCoefMax=[]  ReciprocalOutMin=[]  ReciprocalOutMax=[]  SumDenOutMin=[]  SumDenOutMax=[]  SumNumOutMin=[]  SumNumOutMax=[]  DivideOutMin=[]  DivideOutMax=[]  UdiffTsProdOutMin=[]  UdiffTsProdOutMax=[]  NTsProdOutMin=[]  NTsProdOutMax=[]  UintegralTsProdOutMin=[]  UintegralTsProdOutMax=[]  UngainTsProdOutMin=[]  UngainTsProdOutMax=[]  ClampingZeroOutDataTypeStr=Inherit: Inherit via back propagation  ClampingZeroOutMin=[]  ClampingZeroOutMax=[]  FilterDenConstantOutDataTypeStr=Inherit: Inherit via back propagation  FilterDenConstantOutMin=[]  FilterDenConstantOutMax=[]  PCopyOutDataTypeStr=Inherit: Inherit via back propagation  PCopyOutMin=[]  PCopyOutMax=[]  NCopyOutDataTypeStr=Inherit: Inherit via back propagation  NCopyOutMin=[]  NCopyOutMax=[]  IntegratorContinuousStateAttributes=''  IntegratorStateMustResolveToSignalObject=off  IntegratorRTWStateStorageClass=Auto  FilterContinuousStateAttributes=''  FilterStateMustResolveToSignalObject=off  FilterRTWStateStorageClass=Auto  ParallelPVariant=InternalParameters  IdealPVariant=Disabled  IVariant=InternalParameters  DVariant=InternalParameters  IntegratorVariant=Continuous  SatVariant=Disabled  AWVariant=Passthrough  PCopyVariant=Disabled  TRVariant=Disabled  FdbkBlocksVariant=Forward  IdealPFdbkVariant=Disabled  SatFdbkVariant=Disabled  DerivativeFilterVariant=ContFilter  NVariant=InternalParameters  NCopyVariant=Disabled  FilterICVariant=InternalICsFilter  IntegratorICVariant=InternalICs  ExternalResetVariant=Disabled  TRSumVariant=Passthrough  SumFdbkVariant=Disabled  SumVariant=Sum_PID  TsampFilterVariant=InternalTs  TsampNgainVariant=Passthrough  TsampIntegralVariant=Disabled_SignalSpec  ExternalSaturationOutDataTypeStr=Inherit: Same as second input  DerivativeSourceVariant=ErrorSignal  PreIntVariant=InternalPreInt
  Pitch Limit : Saturate  UpperLimit=pi/3  LowerLimit=-pi/3
  Roll Limit : Saturate  UpperLimit=pi/3  LowerLimit=-pi/3
  Scope : Scope  NumInputPorts=2
      settings: ActiveDisplayYMinimum=-1.96666  ActiveDisplayYMaximum=2.2076  DataLoggingVariableName=ScopeData5
  Subtract2 : Sum  Inputs=+-
  Terminator : Terminator
  Pitch Cmd : Outport
  Roll Cmd : Outport  Port=2
  Yaw Cmd : Outport  Port=3
  Out Bus Element : Outport  Port=4  PortName=Ref  Element=pos
  Out Bus Element1 : Outport  Port=4  PortName=Ref  Element=vel
  Out Bus Element2 : Outport  Port=4  PortName=Ref  Element=roll
  Out Bus Element3 : Outport  Port=4  PortName=Ref  Element=pitch
  Out Bus Element4 : Outport  Port=4  PortName=Ref  Element=yaw
  wires:
  Demux/2 -> Dir R/1
  Mux rpy/1 -> Calculate RBI/1(attitude)
  Demux/1 -> Dir P/1
  Calculate RBI/1(R_BI) -> Matrix Multiply/1
  Mux p/1 -> Subtract2/2
  Subtract2/1 -> Scope/2, PID Controller/1  "Pos Error"
  Err2R/1 -> Roll Limit/1
  In Bus Element7/1 -> Subtract2/1
  Err2P/1 -> Pitch Limit/1
  In Bus Element1/1 -> Mux p/1
  In Bus Element2/1 -> Mux p/2
  In Bus Element3/1 -> Mux p/3
  In Bus Element11/1 -> Mux rpy/3
  In Bus Element8/1 -> Mux rpy/1
  In Bus Element9/1 -> Mux rpy/2
  Pitch Limit/1 -> Out Bus Element3/1, Pitch Cmd/1
  Roll Limit/1 -> Out Bus Element2/1, Roll Cmd/1
  In Bus Element/1 -> Out Bus Element4/1, Yaw Cmd/1
  In Bus Element12/1 -> Out Bus Element/1
  In Bus Element13/1 -> Out Bus Element1/1
  PID Controller/1 -> Matrix Multiply/2
  Demux/3 -> Terminator/1
  Dir P/1 -> Err2P/1
  Dir R/1 -> Err2R/1
  Matrix Multiply/1 -> Filter/1(i)
  Filter/1(o) -> Scope/1, Demux/1
